simulink model "lr4_v20_task2_d0"  (R2023a)
settings: Solver=ode45  StartTime=0  StopTime=1  RelTol=1e-9  AbsTol=1e-11
InitFcn:
  | h=0.01; a=18; p=2; q=4;
settings Model: Creator=theju  LastModifiedBy=theju

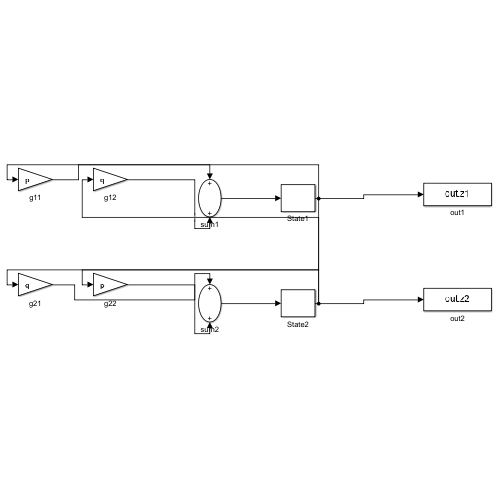
[thumbnail: Simulink's stored preview of the top-level diagram]
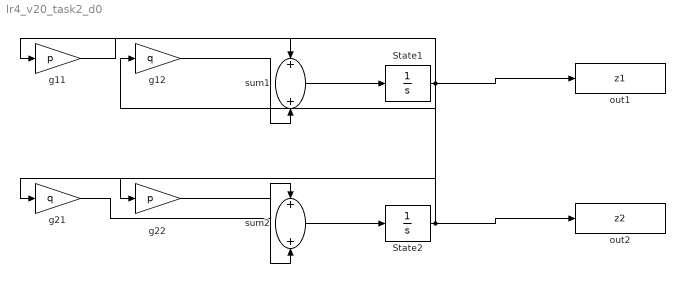
== system lr4_v20_task2_d0 ==
  State1 : Integrator  InitialCondition=3
  State2 : Integrator
  g11 : Gain  Gain=p
  g12 : Gain  Gain=q
  g21 : Gain  Gain=q
  g22 : Gain  Gain=p
  out1 : ToWorkspace  VariableName=z1  SaveFormat=Timeseries  SampleTime=-1
  out2 : ToWorkspace  VariableName=z2  SaveFormat=Timeseries  SampleTime=-1
  sum1 : Sum
  sum2 : Sum
  wires:
  State1/1 -> out1/1, g11/1, g21/1
  State2/1 -> out2/1, g12/1, g22/1
  g11/1 -> sum1/1
  g12/1 -> sum1/2
  sum1/1 -> State1/1
  g21/1 -> sum2/1
  g22/1 -> sum2/2
  sum2/1 -> State2/1
